simulink model "B6_Diag"  (R2022b)
settings: Solver=FixedStepDiscrete  StartTime=0.0  StopTime=20  FixedStep=Ts  RelTol=1e-3
values from neighbouring files (symbols this model uses):
  Ts = 0.01    [build_B2_AutoHeadlamp.m]    (also in build_B3_AHB.m)
undefined symbols (not defined in the file or in its folder): I_NOM, R_OPEN, R_SHORT, T_CONF, T_HEAL, T_INRUSH
settings Model: Creator=LENOVO  LastModifiedBy=LENOVO

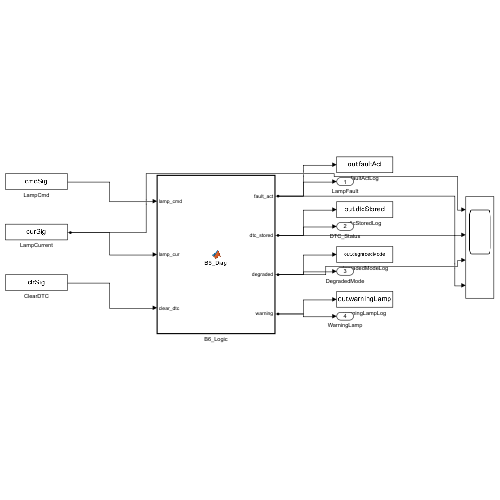
[thumbnail: Simulink's stored preview of the top-level diagram]
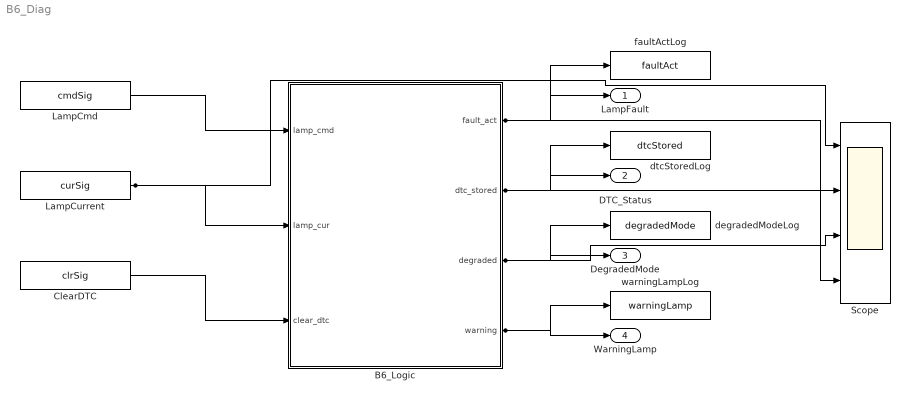
== system B6_Diag ==
  B6_Logic : MATLAB Function  TreatAsAtomicUnit=on
  ClearDTC : FromWorkspace  VariableName=clrSig  SampleTime=Ts  Interpolate=off  OutputAfterFinalValue=Holding final value
  LampCmd : FromWorkspace  VariableName=cmdSig  SampleTime=Ts  Interpolate=off  OutputAfterFinalValue=Holding final value
  LampCurrent : FromWorkspace  VariableName=curSig  SampleTime=Ts  OutputAfterFinalValue=Holding final value
  Scope : Scope  NumInputPorts=4
  degradedModeLog : ToWorkspace  VariableName=degradedMode  SaveFormat=Timeseries  SampleTime=-1
  dtcStoredLog : ToWorkspace  VariableName=dtcStored  SaveFormat=Timeseries  SampleTime=-1
  faultActLog : ToWorkspace  VariableName=faultAct  SaveFormat=Timeseries  SampleTime=-1
  warningLampLog : ToWorkspace  VariableName=warningLamp  SaveFormat=Timeseries  SampleTime=-1
  LampFault : Outport
  DTC_Status : Outport  Port=2
  DegradedMode : Outport  Port=3
  WarningLamp : Outport  Port=4
  wires:
  LampCmd/1 -> B6_Logic/1(lamp_cmd)
  LampCurrent/1 -> B6_Logic/2(lamp_cur), Scope/1
  ClearDTC/1 -> B6_Logic/3(clear_dtc)
  B6_Logic/1(fault_act) -> faultActLog/1, LampFault/1, Scope/2
  B6_Logic/2(dtc_stored) -> dtcStoredLog/1, DTC_Status/1, Scope/4
  B6_Logic/3(degraded) -> degradedModeLog/1, DegradedMode/1, Scope/3
  B6_Logic/4(warning) -> warningLampLog/1, WarningLamp/1

== matlab function B6_Diag/B6_Logic ==
  data: lamp_cmd input; fault_act output; lamp_cur input; clear_dtc input; dtc_stored output; degraded output; warning output; Ts parameter; I_NOM parameter; R_OPEN parameter; R_SHORT parameter; T_INRUSH parameter; T_CONF parameter; T_HEAL parameter
function [fault_act, dtc_stored, degraded, warning] = B6_Diag(lamp_cmd, lamp_cur, clear_dtc, Ts, I_NOM, R_OPEN, R_SHORT, T_INRUSH, T_CONF, T_HEAL)
%#codegen
% B6 - Diagnostic des lampes par mesure du courant
% Lampes : 1 croisement G, 2 croisement D, 3 clignotant G, 4 clignotant D
% dtc_stored : bits 0-3 = circuit ouvert (lampe grillee), bits 4-7 = court-circuit
persistent ton tbo tbs tgood fo fs stored
if isempty(ton)
    ton = zeros(4,1); tbo = zeros(4,1); tbs = zeros(4,1); tgood = zeros(4,1);
    fo = false(4,1); fs = false(4,1); stored = uint16(0);
end
cmd = logical(lamp_cmd(:));  cur = lamp_cur(:);
for i = 1:4
    if cmd(i)
        ton(i) = min(ton(i) + Ts, 100);           % temps depuis l'allumage
    else
        ton(i) = 0;
    end
    if cmd(i) && ton(i) > T_INRUSH + Ts/2         % on ne juge qu'apres le pic d'allumage
        r = cur(i) / I_NOM(i);                    % courant mesure / courant nominal
        bad_open  = r < R_OPEN;                   % < 20 % : lampe grillee (REQ-LSC-22)
        bad_short = r > R_SHORT;                  % > 150 % : court-circuit (REQ-LSC-22)
        if bad_open,  tbo(i) = tbo(i) + Ts; else, tbo(i) = 0; end
        if bad_short, tbs(i) = tbs(i) + Ts; else, tbs(i) = 0; end
        if tbo(i) > T_CONF + Ts/2                 % confirmation 100 ms
            fo(i) = true; stored = bitor(stored, bitshift(uint16(1), i-1));
        end
        if tbs(i) > T_CONF + Ts/2
            fs(i) = true; stored = bitor(stored, bitshift(uint16(1), i+3));
        end
        if ~bad_open && ~bad_short                % mesure correcte : guerison
            tgood(i) = min(tgood(i) + Ts, 100);
            if tgood(i) > T_HEAL + Ts/2
                fo(i) = false; fs(i) = false;     % defaut plus actif (le DTC reste memorise)
            end
        else
            tgood(i) = 0;
        end
    else
        tbo(i) = 0; tbs(i) = 0;                   % lampe eteinte : on ne peut pas juger
    end
end
act = fo | fs;
if clear_dtc                                      % effacement par l'outil de diagnostic
    stored = uint16(0);
    for i = 1:4
        if fo(i), stored = bitor(stored, bitshift(uint16(1), i-1)); end
        if fs(i), stored = bitor(stored, bitshift(uint16(1), i+3)); end
    end
end
fault_act  = act;
dtc_stored = stored;
degraded   = uint8(act(1)) + 2*uint8(act(2));     % 0 aucun, 1 croisement G, 2 croisement D, 3 les deux (REQ-LSC-24)
warning    = any(act);                            % temoin defaut au tableau de bord
